simulink model "rc_transmitter"  (R2026b)
settings: Solver=VariableStepAuto
undefined symbols (not defined in the file or in its folder): P, Ts
libraries: simulink x1
settings Model: Creator=aomar  LastModifiedBy=aomar

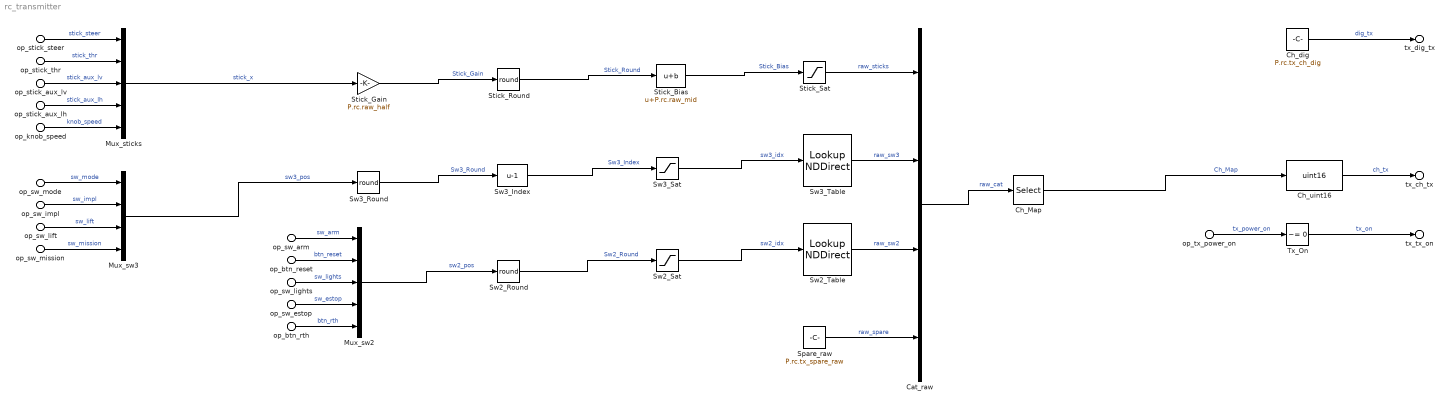
== system rc_transmitter ==
  op_stick_steer : Inport  PortName=op  Element=stick_steer
  op_stick_thr : Inport  PortName=op  Element=stick_thr
  op_stick_aux_lv : Inport  PortName=op  Element=stick_aux_lv
  op_stick_aux_lh : Inport  PortName=op  Element=stick_aux_lh
  op_knob_speed : Inport  PortName=op  Element=knob_speed
  op_sw_mode : Inport  PortName=op  Element=sw_mode
  op_sw_impl : Inport  PortName=op  Element=sw_impl
  op_sw_lift : Inport  PortName=op  Element=sw_lift
  op_sw_mission : Inport  PortName=op  Element=sw_mission
  op_sw_arm : Inport  PortName=op  Element=sw_arm
  op_btn_reset : Inport  PortName=op  Element=btn_reset
  op_sw_lights : Inport  PortName=op  Element=sw_lights
  op_sw_estop : Inport  PortName=op  Element=sw_estop
  op_btn_rth : Inport  PortName=op  Element=btn_rth
  op_tx_power_on : Inport  PortName=op  Element=tx_power_on
  Cat_raw : Concatenate  NumInputs=4
  Ch_Map : Selector  InputPortWidth=P.rc.n_ch  IndexOptions=Index vector (dialog)  Indices=P.rc.tx_perm  OutputSizes=1
  Ch_dig : Constant  Value=P.rc.tx_ch_dig  OutDataTypeStr=boolean  SampleTime=Ts.rc_frame
  Ch_uint16 : DataTypeConversion  OutDataTypeStr=uint16  RndMeth=Round
  Mux_sticks : Mux  Inputs=5
  Mux_sw2 : Mux  Inputs=5
  Mux_sw3 : Mux
  Spare_raw : Constant  Value=P.rc.tx_spare_raw  SampleTime=Ts.rc_frame
  Stick_Bias : Bias  Bias=P.rc.raw_mid  SaturateOnIntegerOverflow=off
  Stick_Gain : Gain  Gain=P.rc.raw_half
  Stick_Round : Rounding  Operator=round
  Stick_Sat : Saturate  UpperLimit=P.rc.raw_max  LowerLimit=P.rc.raw_min
  Sw2_Round : Rounding  Operator=round
  Sw2_Sat : Saturate  UpperLimit=numel(P.rc.raw_sw2)-1  LowerLimit=0
  Sw2_Table : LookupNDDirect  NumberOfTableDimensions=1  Table=P.rc.raw_sw2  DiagnosticForOutOfRangeInput=Error
  Sw3_Index : Bias  Bias=-1  SaturateOnIntegerOverflow=off
  Sw3_Round : Rounding  Operator=round
  Sw3_Sat : Saturate  UpperLimit=numel(P.rc.raw_sw3)-1  LowerLimit=0
  Sw3_Table : LookupNDDirect  NumberOfTableDimensions=1  Table=P.rc.raw_sw3  DiagnosticForOutOfRangeInput=Error
  Tx_On : simulink/Logic and Bit Operations/Compare To Constant  relop=~=  const=0  OutDataTypeStr=boolean
  tx_ch_tx : Outport  PortName=tx  Element=ch_tx
  tx_dig_tx : Outport  PortName=tx  Element=dig_tx
  tx_tx_on : Outport  PortName=tx  Element=tx_on
  wires:
  op_stick_steer/1 -> Mux_sticks/1  "stick_steer"
  op_stick_thr/1 -> Mux_sticks/2  "stick_thr"
  op_stick_aux_lv/1 -> Mux_sticks/3  "stick_aux_lv"
  op_stick_aux_lh/1 -> Mux_sticks/4  "stick_aux_lh"
  op_knob_speed/1 -> Mux_sticks/5  "knob_speed"
  op_sw_mode/1 -> Mux_sw3/1  "sw_mode"
  op_sw_impl/1 -> Mux_sw3/2  "sw_impl"
  op_sw_lift/1 -> Mux_sw3/3  "sw_lift"
  op_sw_mission/1 -> Mux_sw3/4  "sw_mission"
  Mux_sticks/1 -> Stick_Gain/1  "stick_x"
  Mux_sw3/1 -> Sw3_Round/1  "sw3_pos"
  op_sw_arm/1 -> Mux_sw2/1  "sw_arm"
  op_btn_reset/1 -> Mux_sw2/2  "btn_reset"
  op_sw_lights/1 -> Mux_sw2/3  "sw_lights"
  op_sw_estop/1 -> Mux_sw2/4  "sw_estop"
  op_btn_rth/1 -> Mux_sw2/5  "btn_rth"
  Mux_sw2/1 -> Sw2_Round/1  "sw2_pos"
  Stick_Gain/1 -> Stick_Round/1  "Stick_Gain"
  Sw3_Round/1 -> Sw3_Index/1  "Sw3_Round"
  Stick_Round/1 -> Stick_Bias/1  "Stick_Round"
  Sw2_Round/1 -> Sw2_Sat/1  "Sw2_Round"
  Sw3_Index/1 -> Sw3_Sat/1  "Sw3_Index"
  Sw3_Sat/1 -> Sw3_Table/1  "sw3_idx"
  Sw2_Sat/1 -> Sw2_Table/1  "sw2_idx"
  Stick_Bias/1 -> Stick_Sat/1  "Stick_Bias"
  Stick_Sat/1 -> Cat_raw/1  "raw_sticks"
  Spare_raw/1 -> Cat_raw/4  "raw_spare"
  Sw3_Table/1 -> Cat_raw/2  "raw_sw3"
  Sw2_Table/1 -> Cat_raw/3  "raw_sw2"
  Cat_raw/1 -> Ch_Map/1  "raw_cat"
  Ch_Map/1 -> Ch_uint16/1  "Ch_Map"
  op_tx_power_on/1 -> Tx_On/1  "tx_power_on"
  Ch_dig/1 -> tx_dig_tx/1  "dig_tx"
  Tx_On/1 -> tx_tx_on/1  "tx_on"
  Ch_uint16/1 -> tx_ch_tx/1  "ch_tx"
